simulink model "Water_Tank"  (R2023a)
settings: Solver=VariableStepAuto  StartTime=0.0  StopTime=200  RelTol=1e-3
values from neighbouring files (symbols this model uses):
  Kd_init = 1    [comparison_code.m]    (also in evaluation_code.m)
  Ki_init = 2.5    [comparison_code.m]    (also in evaluation_code.m)
  Kp_init = 5    [comparison_code.m]    (also in evaluation_code.m)
undefined symbols (not defined in the file or in its folder): DiscIntNeverNeededParam, start_h, target_h
libraries: simulink x3, rllib x1, slpidlib x1
settings Model: Creator=HP  LastModifiedBy=HP

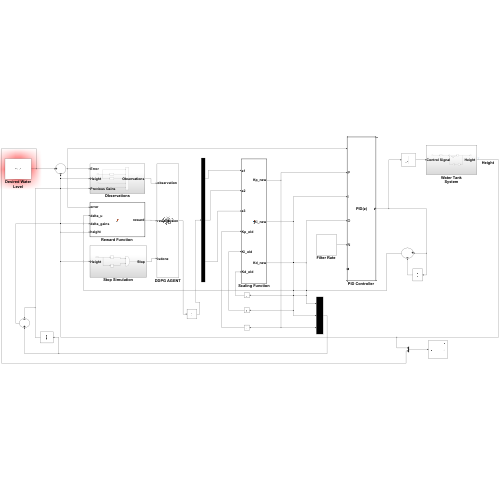
[thumbnail: Simulink's stored preview of the top-level diagram]
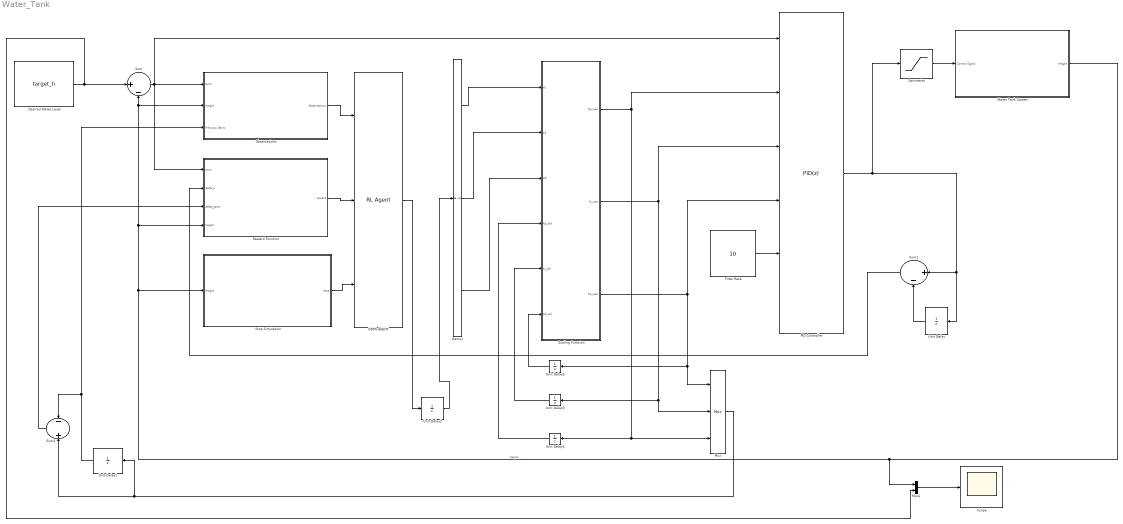
== system Water_Tank ==
  DDPG AGENT : rllib/RL Agent  Agent=DDPG_AGENT_2000  ExternalActionAsInput=off  ProvideLastAction=off  ProvideCumRwd=off  TreatAsDirectFeedthrough=on  UseStrictObservationDataTypes=off
  Demux : Demux  Outputs=3
  Desired Water Level : Constant  Value=target_h
  "Filter Rate " : Constant  Value=10
  Mux : Mux  Inputs=3
  Mux1 : Mux  Inputs=2
  Observations : Subsystem
  "PID Controller " : slpidlib/PID Controller  Controller=PID  Form=Parallel  TimeDomain=Discrete-time  UseExternalTs=off  SampleTime=1  IntegratorMethod=Backward Euler  FilterMethod=Backward Euler  ControllerParametersSource=external  P=1  I=1  UseKiTs=off  D=0  N=100  UseFilter=on  TunerSelectOption=Transfer Function Based (PID Tuner App)  ZeroCross=off  InitialConditionSource=internal  InitialConditionForIntegrator=0  InitialConditionForFilter=0  DifferentiatorICPrevScaledInput=0  ExternalReset=level  TrackingMode=off  Kt=1  LimitOutput=on  SatLimitsSource=internal  UpperSaturationLimit=10  LowerSaturationLimit=0  LinearizeAsGain=on  AntiWindupMode=clamping  Kb=1  LimitIntegrator=off  UpperIntegratorSaturationLimit=inf  LowerIntegratorSaturationLimit=-inf  RndMeth=Zero  POutMin=[]  POutMax=[]  IOutMin=[]  IOutMax=[]  DOutMin=[]  DOutMax=[]  NOutMin=[]  NOutMax=[]  SumOutMin=[]  SumOutMax=[]  SaturationOutMin=[]  SaturationOutMax=[]  PParamMin=[]  PParamMax=[]  IParamMin=[]  IParamMax=[]  DParamMin=[]  DParamMax=[]  NParamMin=[]  NParamMax=[]  KbParamMin=[]  KbParamMax=[]  KtParamMin=[]  KtParamMax=[]  KbOutMin=[]  KbOutMax=[]  KtOutMin=[]  KtOutMax=[]  IntegratorOutMin=[]  IntegratorOutMax=[]  FilterOutMin=[]  FilterOutMax=[]  SumI1OutMin=[]  SumI1OutMax=[]  SumI2OutMin=[]  SumI2OutMax=[]  SumI3OutMin=[]  SumI3OutMax=[]  SumI4OutMin=[]  SumI4OutMax=[]  SumDOutMin=[]  SumDOutMax=[]  DifferentiatorOutMin=[]  DifferentiatorOutMax=[]  FilterDiffOutCoefMin=[]  FilterDiffOutCoefMax=[]  ReciprocalOutMin=[]  ReciprocalOutMax=[]  SumDenOutMin=[]  SumDenOutMax=[]  SumNumOutMin=[]  SumNumOutMax=[]  DivideOutMin=[]  DivideOutMax=[]  UdiffTsProdOutMin=[]  UdiffTsProdOutMax=[]  NTsProdOutMin=[]  NTsProdOutMax=[]  UintegralTsProdOutMin=[]  UintegralTsProdOutMax=[]  UngainTsProdOutMin=[]  UngainTsProdOutMax=[]  ClampingZeroOutDataTypeStr=Inherit: Inherit via back propagation  ClampingZeroOutMin=[]  ClampingZeroOutMax=[]  FilterDenConstantOutDataTypeStr=Inherit: Inherit via back propagation  FilterDenConstantOutMin=[]  FilterDenConstantOutMax=[]  PCopyOutDataTypeStr=Inherit: Inherit via back propagation  PCopyOutMin=[]  PCopyOutMax=[]  NCopyOutDataTypeStr=Inherit: Inherit via back propagation  NCopyOutMin=[]  NCopyOutMax=[]  IntegratorContinuousStateAttributes=''  IntegratorStateMustResolveToSignalObject=off  IntegratorRTWStateStorageClass=Auto  FilterContinuousStateAttributes=''  FilterStateMustResolveToSignalObject=off  FilterRTWStateStorageClass=Auto  ParallelPVariant=ExternalParameters  IdealPVariant=Disabled  IVariant=ExternalParameters  DVariant=ExternalParameters  IntegratorVariant=Discrete  SatVariant=Enabled  AWVariant=DiscClampingParallel  PCopyVariant=Disabled  TRVariant=Disabled  FdbkBlocksVariant=Feedback  IdealPFdbkVariant=Passthrough  SatFdbkVariant=Passthrough  DerivativeFilterVariant=BackwardEulerFilter  NVariant=ExternalParameters  NCopyVariant=ExternalParameters  FilterICVariant=InternalICsFilter  IntegratorICVariant=InternalICs  ExternalResetVariant=ExternalReset  TRSumVariant=Passthrough  SumFdbkVariant=Enabled  SumVariant=Sum_PID  TsampFilterVariant=InternalTs  TsampNgainVariant=Passthrough  TsampIntegralVariant=Disabled_SignalSpec  ExternalSaturationOutDataTypeStr=Inherit: Same as second input
  "Reward Function " : MATLAB Function  TreatAsAtomicUnit=on
  Saturation : Saturate  UpperLimit=10  LowerLimit=0
  Scaling Function : MATLAB Function  TreatAsAtomicUnit=on
  Scope : Scope
  Stop Simulation : Subsystem
  Sum : Sum  Inputs=|+-
  Sum1 : Sum  Inputs=|+-
  Sum2 : Sum  Inputs=-+
  Unit Delay : UnitDelay  HasFrameUpgradeWarning=on
  Unit Delay1 : UnitDelay  HasFrameUpgradeWarning=on
  Unit Delay2 : UnitDelay  HasFrameUpgradeWarning=on
  Unit Delay3 : UnitDelay  InitialCondition=Ki_init  HasFrameUpgradeWarning=on
  Unit Delay4 : UnitDelay  InitialCondition=Kp_init  HasFrameUpgradeWarning=on
  Unit Delay5 : UnitDelay  InitialCondition=Kd_init  HasFrameUpgradeWarning=on
  Water Tank System : Subsystem
  wires:
  Water Tank System/1("Height ") -> Mux1/1, Sum/2, Observations/2(Height), "Reward Function "/4(height), Stop Simulation/1(Height)  "Height"
  Desired Water Level/1 -> Sum/1, Mux1/2
  Sum/1 -> "PID Controller "/1, Observations/1(Error), "Reward Function "/1(error)
  "Filter Rate "/1 -> "PID Controller "/5
  Demux/1 -> Scaling Function/1(a1)
  Demux/2 -> Scaling Function/2(a2)
  Demux/3 -> Scaling Function/3(a3)
  Scaling Function/1(Kp_new) -> "PID Controller "/2, Unit Delay4/1, Mux/3
  Scaling Function/2(Ki_new) -> "PID Controller "/3, Mux/2, Unit Delay3/1
  Scaling Function/3(Kd_new) -> "PID Controller "/4, Mux/1, Unit Delay5/1
  Sum1/1 -> "Reward Function "/2(delta_u)
  Sum2/1 -> "Reward Function "/3(delta_gains)
  Mux/1 -> Sum2/2, Unit Delay1/1
  "PID Controller "/1 -> Unit Delay/1, Sum1/1, Saturation/1
  Unit Delay1/1 -> Observations/3(Previous Gains), Sum2/1
  Unit Delay2/1 -> Demux/1
  Mux1/1 -> Scope/1
  Unit Delay/1 -> Sum1/2
  Unit Delay4/1 -> Scaling Function/4(Kp_old)
  Unit Delay5/1 -> Scaling Function/6(Kd_old)
  Unit Delay3/1 -> Scaling Function/5(Ki_old)
  Observations/1(Observations) -> DDPG AGENT/1
  "Reward Function "/1(reward) -> DDPG AGENT/2
  Stop Simulation/1("Stop ") -> DDPG AGENT/3
  DDPG AGENT/1 -> Unit Delay2/1
  Saturation/1 -> Water Tank System/1("Control Signal ")

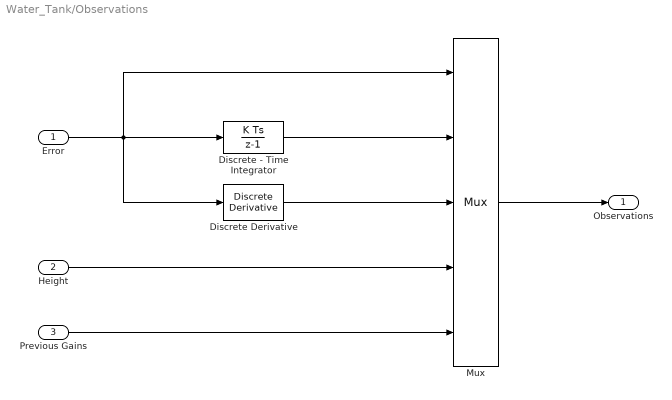
== system Water_Tank/Observations ==
  Error : Inport
  Height : Inport  Port=2
  Previous Gains : Inport  Port=3
  "Discrete - Time Integrator " : DiscreteIntegrator  ICPrevOutput=DiscIntNeverNeededParam  ICPrevScaledInput=DiscIntNeverNeededParam
  "Discrete Derivative " : simulink/Discrete/Discrete Derivative  gainval=1.0  ICPrevScaledInput=0.0  OutMin=[]  OutMax=[]  OutDataType=fixdt(1, 16)  OutScaling=2^-10  DoSatur=off
  Mux : Mux  Inputs=5
  Observations : Outport
  wires:
  Error/1 -> Mux/1, "Discrete Derivative "/1, "Discrete - Time Integrator "/1
  "Discrete Derivative "/1 -> Mux/3
  Height/1 -> Mux/4
  Mux/1 -> Observations/1
  "Discrete - Time Integrator "/1 -> Mux/2
  Previous Gains/1 -> Mux/5

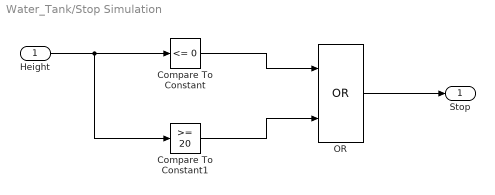
== system Water_Tank/Stop Simulation ==
  Height : Inport
  Compare To Constant : simulink/Logic and Bit Operations/Compare To Constant  relop=<=  const=0  OutDataTypeStr=boolean
  Compare To Constant1 : simulink/Logic and Bit Operations/Compare To Constant  relop=>=  const=20  OutDataTypeStr=boolean
  OR : Logic  Operator=OR  IconShape=distinctive  AllPortsSameDT=off  OutDataTypeStr=boolean
  "Stop " : Outport
  wires:
  Height/1 -> Compare To Constant1/1, Compare To Constant/1
  Compare To Constant/1 -> OR/1
  Compare To Constant1/1 -> OR/2
  OR/1 -> "Stop "/1

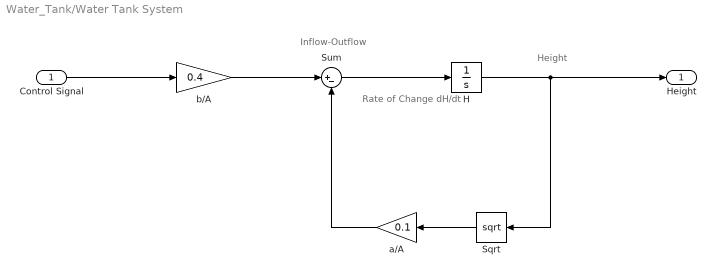
== system Water_Tank/Water Tank System ==
  note: Inflow-Outflow
  note: Rate of Change
      | dH/dt
  note: Height
  "Control Signal " : Inport
  H : Integrator  InitialCondition=start_h  LimitOutput=on  UpperSaturationLimit=20  LowerSaturationLimit=0.001
  Sqrt : Sqrt
  Sum : Sum  Inputs=|+-
  a/A : Gain  Gain=0.1
  b/A : Gain  Gain=0.4
  "Height " : Outport
  wires:
  Sum/1 -> H/1
  "Control Signal "/1 -> b/A/1
  b/A/1 -> Sum/1
  H/1 -> "Height "/1, Sqrt/1
  a/A/1 -> Sum/2
  Sqrt/1 -> a/A/1

== matlab function Water_Tank/Reward Function  ==
  data: error input; delta_u input; delta_gains input; reward output; height input
function reward = fcn(error, delta_u, delta_gains, height)

    h_max   = 20;
    abs_err = abs(error);
    delta   = 1.0;

    % ERROR PENALTY — Huber style, no normalization
    if abs_err <= delta
        penalty_error = abs_err;
    else
        penalty_error = (abs_err^2 + delta^2) / (2 * delta);
    end
    penalty_error = 0.08 * penalty_error;

    % APPROACH VELOCITY PENALTY
    % Penalizes large control changes (primary oscillation killer)

    rate = delta_u / 10;
    penalty_rate = 0.25 * rate^2;

    % DIRECTIONAL OVERSHOOT PENALTY
    % Fires when height has passed target in any direction
    
    overshoot_penalty = 0;
    if (error > 0 && delta_u < -0.3) || (error < 0 && delta_u > 0.3)
        overshoot_penalty = 0.2 * abs_err;
    end

    % CONTROL EFFORT PENALTY — unchanged
    penalty_effort = 0.005 * (delta_u / 10)^2;

    % GAIN FREEZING PENALTY
    % Activates aggressively within 1m of target
    
    proximity = max(0, 1 - abs_err / 2);
    w3 = 0.8 * proximity^3;
    penalty_gains = w3 * sum(delta_gains.^2);

    % BASE REWARD
    reward = -(penalty_error + penalty_rate + overshoot_penalty + ...
               penalty_effort + penalty_gains);

    % TIERED SETTLING BONUS
    % Agent must be genuinely still

    rate_mag = abs(delta_u) / 10;
    if abs_err < 0.05 && rate_mag < 0.01
        reward = reward + 4.0;
    elseif abs_err < 0.15 && rate_mag < 0.03
        reward = reward + 2.0;
    elseif abs_err < 0.4 && rate_mag < 0.10
        reward = reward + 0.4;
    end

    % OUT OF BOUNDS
    if height <= 0 || height >= h_max
        reward = reward - 5;
    end

end

== matlab function Water_Tank/Scaling Function ==
  data: Kp_new output; a1 input; a2 input; a3 input; Ki_new output; Kd_new output; Kp_old input; Ki_old input; Kd_old input
function [Kp_new, Ki_new, Kd_new] = fcn(a1, a2, a3, Kp_old, Ki_old, Kd_old)
    delta_Kp = a1 * 0.3;   
    delta_Ki = a2 * 0.3;     
    delta_Kd = a3 * 0.05;   

    Kp_new = min(max(Kp_old + delta_Kp, 0), 10);
    Ki_new = min(max(Ki_old + delta_Ki, 0), 20);
    Kd_new = min(max(Kd_old + delta_Kd, 0), 2);
end
